simulink model "FMS"  (R2018b)
settings: configuration reference "fms_config" (kept outside this file)
values from neighbouring files (symbols this model uses):
  FMS_EXPORT = Simulink.Parameter(FMS_EXPORT_VALUE)    [fms_model_init.m]
  FMS_PARAM = Simulink.Parameter(FMS_PARAM_VALUE)    [fms_model_init.m]
undefined symbols (not defined in the file or in its folder): actuator_cmd, ax_cmd, ay_cmd, az_cmd, cmd_mask, ControlMode, ctrl_mode, DiscIntNeverNeededParam, ext_state, FMS_Cmd, FMS_CONST, home, mode, p_cmd, phi_cmd, PilotMode, psi_rate_cmd, q_cmd, r_cmd, reset, state, status, theta_cmd, throttle_cmd, timestamp, u_cmd, v_cmd, VehicleState, VehicleStatus, VTOLState, w_cmd, wp_consume, wp_current
libraries: simulink x141, FMT_Model_Lib x120, hdlsllib x13
(part 4 of 12)

== system FMS/FMS Commander/Commander/Arm/MC_Mode/SubMode/Takeoff/Climb Speed ==
  FMS_In : Inport
  Abs : Abs
  Abs1 : Abs
  Bus Selector : BusSelector  OutputSignals=INS_Out.h_R
  Bus Selector1 : BusSelector  OutputSignals=Cmd_In.cur_waypoint
  Bus Selector2 : BusSelector  OutputSignals=Cmd_In.sp_waypoint
  Compare To Constant : simulink/Logic and Bit Operations/Compare To Constant  relop=>  const=2.0  OutDataTypeStr=boolean
  Compare To Constant1 : simulink/Logic and Bit Operations/Compare To Constant  relop=>  const=2.0  OutDataTypeStr=boolean
  Gain : Gain  Gain=0.5
  Logical Operator : Logic  AllPortsSameDT=off  OutDataTypeStr=boolean
  Selector : Selector  InputPortWidth=3  IndexOptions=Index vector (dialog)  Indices=3  OutputSizes=1
  Selector1 : Selector  InputPortWidth=3  IndexOptions=Index vector (dialog)  Indices=3  OutputSizes=1
  Sum : Sum  Inputs=|+-
  Sum1 : Sum  Inputs=|+-
  Switch : Switch  Criteria=u2 ~= 0  Threshold=2
  TD : Subsystem
  Takeoff_Speed : Constant  Value=-FMS_PARAM.TAKEOFF_SPEED  OutDataTypeStr=Inherit: Inherit via back propagation
  w_cmd_mPs : Outport
  wires:
  Takeoff_Speed/1 -> Gain/1, Switch/1
  Sum/1 -> Abs/1
  Bus Selector/1 -> Sum1/2, Sum/1  "<h_R>"
  Switch/1 -> TD/1(v)
  FMS_In/1 -> Bus Selector2/1, Bus Selector/1, Bus Selector1/1
  Selector/1 -> Sum/2
  Bus Selector1/1 -> Selector/1  "<cur_waypoint>"
  Abs/1 -> Compare To Constant1/1
  Bus Selector2/1 -> Selector1/1  "<sp_waypoint>"
  Selector1/1 -> Sum1/1
  Sum1/1 -> Abs1/1
  Abs1/1 -> Compare To Constant/1
  Compare To Constant/1 -> Logical Operator/1
  Compare To Constant1/1 -> Logical Operator/2
  Logical Operator/1 -> Switch/2
  TD/1(v1) -> w_cmd_mPs/1
  Gain/1 -> Switch/3

== system FMS/FMS Commander/Commander/Arm/MC_Mode/SubMode/Takeoff/Track Position ==
  FMS_In : Inport
  Bus Selector : BusSelector  OutputSignals=INS_Out.psi
  Bus_Selection : Subsystem
  Constant : Constant  Value=0  OutDataTypeStr=Inherit: Inherit via back propagation
  Gain2 : Gain  Gain=FMS_PARAM.XY_P  OutDataTypeStr=single
  Multiply : Product  Multiplication=Matrix(*)
  Mux : Mux  Inputs=2
  Psi To DCM : FMT_Model_Lib/Transformation/Psi To DCM
      settings: SourceProductName=FMT Toolbox
  Saturation1 : Saturate  UpperLimit=FMS_PARAM.VEL_XY_LIM/5  LowerLimit=-FMS_PARAM.VEL_XY_LIM/5
  Selector : Selector  InputPortWidth=3  IndexOptions=Index vector (dialog)  Indices=[1 2]  OutputSizes=1
  Sum : Sum  Inputs=-+|
  Target Position : Subsystem
  uv_cmd_mPs : Outport
  wires:
  Saturation1/1 -> uv_cmd_mPs/1
  Bus Selector/1 -> Psi To DCM/1  "<psi>"
  Selector/1 -> Gain2/1
  Mux/1 -> Multiply/2
  Multiply/1 -> Selector/1
  Psi To DCM/1 -> Multiply/1  "M_CO"
  Constant/1 -> Mux/2
  FMS_In/1 -> Bus Selector/1, Target Position/1(FMS_In), Bus_Selection/1(FMS_In)
  Sum/1 -> Mux/1  "xy_err_R"
  Bus_Selection/1(xy_est_R) -> Sum/1  "xy_est_R"
  Gain2/1 -> Saturation1/1
  Target Position/1(xy_cmd_R) -> Sum/2

== system FMS/FMS Commander/Commander/Arm/BackwardTrans_Mode/Position Command/Controller/Hold Control/Fly_Direction ==
  FMS_In : Inport
  Bus Selector2 : BusSelector  OutputSignals=INS_Out.vn,INS_Out.ve,INS_Out.vd
  Bus Selector3 : BusSelector  OutputSignals=INS_Out.quat
  Multiply : Product  Multiplication=Matrix(*)
  Mux : Mux  Inputs=3
  Quaternion To DCM : FMT_Model_Lib/Quaternion/Quaternion To DCM
      settings: SourceProductName=FMT Toolbox
  Selector : Selector  InputPortWidth=3  IndexOptions=Index vector (dialog)  Indices=1  OutputSizes=1
  Sign : Signum
  sign : Outport
  wires:
  Bus Selector3/1 -> Quaternion To DCM/1  "<quat>"
  Multiply/1 -> Selector/1
  Bus Selector2/3 -> Mux/3  "<vd>"
  FMS_In/1 -> Bus Selector3/1, Bus Selector2/1
  Sign/1 -> sign/1
  Mux/1 -> Multiply/2
  Quaternion To DCM/1 -> Multiply/1
  Bus Selector2/2 -> Mux/2  "<ve>"
  Bus Selector2/1 -> Mux/1  "<vn>"
  Selector/1 -> Sign/1  "Vu"

== system FMS/FMS Commander/Commander/Arm/BackwardTrans_Mode/Position Command/Controller/Hold Control/L1_Reference_WP ==
  c : Inport
  p_0 : Inport  Port=2
  n : Inport  Port=3
  L1 : Inport  Port=4
  Compare To Zero : simulink/Logic and Bit Operations/Compare To Zero  relop=>  OutDataTypeStr=boolean
  OutRegionRefWP : MATLAB Function  TreatAsAtomicUnit=on
  SearchL1RefWP : MATLAB Function  TreatAsAtomicUnit=on
  Switch : Switch  Criteria=u2 > Threshold
  L1_WP : Outport
  wires:
  c/1 -> OutRegionRefWP/1(c), SearchL1RefWP/1(c)
  p_0/1 -> OutRegionRefWP/2(p0), SearchL1RefWP/2(p0)
  n/1 -> OutRegionRefWP/3(n), SearchL1RefWP/3(n)
  L1/1 -> SearchL1RefWP/4(L1)
  SearchL1RefWP/1(P) -> Switch/1
  SearchL1RefWP/2(t) -> Compare To Zero/1
  Compare To Zero/1 -> Switch/2
  OutRegionRefWP/1(P) -> Switch/3
  Switch/1 -> L1_WP/1

== system FMS/FMS Commander/Commander/Arm/BackwardTrans_Mode/Position Command/Controller/Hold Control/Lateral_Acceleration ==
  p_vehicle : Inport
  L1_WP : Inport  Port=2
  L1 : Inport  Port=3
  Vg : Inport  Port=4
  L1_Lateral_Acceleration : Subsystem
  Subtract : Sum  Inputs=+-
  ay_cmd_mPs2 : Outport
  wires:
  L1_WP/1 -> Subtract/1
  p_vehicle/1 -> Subtract/2
  L1/1 -> L1_Lateral_Acceleration/1(L1)
  Vg/1 -> L1_Lateral_Acceleration/2(Vg)
  Subtract/1 -> L1_Lateral_Acceleration/3(l1_path)
  L1_Lateral_Acceleration/1(l1_a_cmd) -> ay_cmd_mPs2/1

== system FMS/FMS Commander/Commander/Arm/BackwardTrans_Mode/Position Command/Controller/Hold Control/Path_Ray ==
  note: p(t) = p0 + t*n
  FMS_In : Inport
  Bus Selector1 : BusSelector  OutputSignals=INS_Out.x_R,INS_Out.y_R
  Bus Selector2 : BusSelector  OutputSignals=INS_Out.vn,INS_Out.ve
  Bus Selector3 : BusSelector  Commented=on  OutputSignals=INS_Out.psi
  Constant : Constant  Commented=on  Value=[1;0;0]  VectorParams1D=off  OutDataTypeStr=single
  Multiply : Product  Commented=on  Multiplication=Matrix(*)
  Mux : Mux  Inputs=2
  Mux1 : Mux  Inputs=2
  Psi To DCM : FMT_Model_Lib/Transformation/Psi To DCM  Commented=on
      settings: SourceProductName=FMT Toolbox
  Selector : Selector  Commented=on  InputPortWidth=3  IndexOptions=Index vector (dialog)  Indices=[1 2]  OutputSizes=1
  Terminator : Terminator  Commented=on
  Transpose : Math  Commented=on  Operator=transpose  SaturateOnIntegerOverflow=on
  Vector Normalize : FMT_Model_Lib/Math/Vector Normalize
      settings: SourceProductName=FMT Toolbox
  start_vel : Delay  DelayLength=1  InitialConditionSource=Input port
      settings: InputPortMap=u0,p4
  start_wp : Delay  DelayLength=1  InitialConditionSource=Input port
      settings: InputPortMap=u0,p4
  p_vehicle : Outport
  p_0 : Outport  Port=2
  n : Outport  Port=3
  wires:
  Bus Selector2/2 -> Mux1/2  "<ve>"
  Bus Selector1/2 -> Mux/2  "<y_R>"
  Mux/1 -> p_vehicle/1, start_wp/2
  start_wp/1 -> p_0/1, start_wp/1
  Bus Selector1/1 -> Mux/1  "<x_R>"
  start_vel/1 -> Vector Normalize/1, start_vel/1
  Bus Selector2/1 -> Mux1/1  "<vn>"
  Vector Normalize/1 -> n/1
  FMS_In/1 -> Bus Selector3/1, Bus Selector2/1, Bus Selector1/1
  Mux1/1 -> start_vel/2
  Bus Selector3/1 -> Psi To DCM/1  "<psi>"
  Psi To DCM/1 -> Transpose/1
  Transpose/1 -> Multiply/1
  Constant/1 -> Multiply/2
  Multiply/1 -> Selector/1
  Selector/1 -> Terminator/1

== system FMS/FMS Commander/Commander/Arm/BackwardTrans_Mode/Position Command/Controller/Hold Control/Velocity_Controller ==
  FMS_In : Inport
  Bus Selector : BusSelector  OutputSignals=INS_Out
  Constant : Constant  Value=0  OutDataTypeStr=Inherit: Inherit via back propagation
  Error : Subsystem
  PID_Controller : Subsystem
  ay_cmd_B_rad : Outport
  wires:
  FMS_In/1 -> Bus Selector/1
  Error/1(v_err_C_mPs) -> PID_Controller/1(uv_err_C_mPs)
  PID_Controller/1(accel_cmd_C) -> ay_cmd_B_rad/1
  Bus Selector/1 -> Error/1(INS_Out)  "<INS_Out>"
  Constant/1 -> PID_Controller/2(reset)

== system FMS/FMS Commander/Commander/Arm/BackwardTrans_Mode/Position Command/Controller/Move Control/DeadZone1 ==
  u : Inport
  Dead Zone : DeadZone  LowerValue=-th  UpperValue=th  SaturateOnIntegerOverflow=on
  Gain : Gain  Gain=1/(1-th)
  y : Outport
  wires:
  u/1 -> Dead Zone/1
  Dead Zone/1 -> Gain/1
  Gain/1 -> y/1

== system FMS/FMS Commander/Commander/Arm/BackwardTrans_Mode/Position Command/Controller/Move Control/TD ==
  v : Inport
  Integrator : DiscreteIntegrator  SampleTime=-1  ICPrevOutput=DiscIntNeverNeededParam  ICPrevScaledInput=DiscIntNeverNeededParam
  Integrator1 : DiscreteIntegrator  SampleTime=-1  ICPrevOutput=DiscIntNeverNeededParam  ICPrevScaledInput=DiscIntNeverNeededParam
  Subtract : Sum  Inputs=+-
  "fhan " : Subsystem  mask{r0=6*9.806, h0=0.05}
      mask DialogControl ParameterGroupVar Prompt: fhan(v1,v2,r0,h0)
  v1 : Outport
  wires:
  "fhan "/1(fhan) -> Integrator/1
  Subtract/1 -> "fhan "/1(v1)
  Integrator/1 -> Integrator1/1, "fhan "/2(v2)  "v2"
  v/1 -> Subtract/2
  Integrator1/1 -> Subtract/1, v1/1

== system FMS/FMS Commander/Commander/Arm/FW_Mode/Assist/Altitude/Altitude Command/Controller ==
  motion_state : Inport
  In Bus Element : Inport  Port=2  PortName=FMS_In
  In Bus Element1 : Inport  Port=2  PortName=FMS_In
  Hold Control : Subsystem  TreatAsAtomicUnit=on
  Merge : Merge
  Move Control : Subsystem  TreatAsAtomicUnit=on
  Saturation1 : Saturate  UpperLimit=FMS_PARAM.FW_VEL_Z_LIM  LowerLimit=-FMS_PARAM.FW_VEL_Z_LIM
  Switch Case : SwitchCase  CaseConditions={MotionState.Hold, [MotionState.Brake, MotionState.Move]}  ShowDefaultCase=off
  TD : Subsystem
  w_cmd_mPs : Outport
  wires:
  Move Control/1(w_cmd_mPs) -> Merge/2
  Hold Control/1(w_cmd_mPs) -> Merge/1
  In Bus Element/1 -> Hold Control/1(FMS_In)
  Switch Case/2 -> Move Control/Action
  Switch Case/1 -> Hold Control/Action
  motion_state/1 -> Switch Case/1
  Saturation1/1 -> TD/1(v)
  Merge/1 -> Saturation1/1
  In Bus Element1/1 -> Move Control/1(FMS_In)
  TD/1(v1) -> w_cmd_mPs/1

== system FMS/FMS Commander/Commander/Arm/FW_Mode/Assist/Altitude/Altitude Command/Detect Movement ==
  FMS_In : Inport
  Abs : Abs
  Abs1 : Abs
  Bus Selector : BusSelector  OutputSignals=Pilot_Cmd.stick_pitch,INS_Out.vd
  Compare To Constant : simulink/Logic and Bit Operations/Compare To Constant  relop=>  const=FMS_PARAM.PITCH_DZ  OutDataTypeStr=boolean
  Motion Status : Stateflow chart  TreatAsAtomicUnit=on
  motion_state : Outport
  wires:
  FMS_In/1 -> Bus Selector/1
  Abs1/1 -> Compare To Constant/1
  Motion Status/1(state) -> motion_state/1
  Compare To Constant/1 -> Motion Status/1(motion_req)
  Abs/1 -> Motion Status/2(speed)
  Bus Selector/1 -> Abs1/1  "<stick_pitch>"
  Bus Selector/2 -> Abs/1  "<vd>"

== system FMS/FMS Commander/Commander/Arm/FW_Mode/Assist/Altitude/Attitude Command/DeadZone ==
  u : Inport
  Dead Zone : DeadZone  LowerValue=-th  UpperValue=th  SaturateOnIntegerOverflow=on
  Gain : Gain  Gain=1/(1-th)
  y : Outport
  wires:
  Gain/1 -> y/1
  Dead Zone/1 -> Gain/1
  u/1 -> Dead Zone/1

== system FMS/FMS Commander/Commander/Arm/FW_Mode/Assist/Altitude/Attitude Command/TD ==
  v : Inport
  Integrator : DiscreteIntegrator  SampleTime=-1  ICPrevOutput=DiscIntNeverNeededParam  ICPrevScaledInput=DiscIntNeverNeededParam
  Integrator1 : DiscreteIntegrator  SampleTime=-1  ICPrevOutput=DiscIntNeverNeededParam  ICPrevScaledInput=DiscIntNeverNeededParam
  Subtract : Sum  Inputs=+-
  "fhan " : Subsystem  mask{r0=4*pi, h0=0.04}
      mask DialogControl ParameterGroupVar Prompt: fhan(v1,v2,r0,h0)
  v1 : Outport
  wires:
  "fhan "/1(fhan) -> Integrator/1
  Subtract/1 -> "fhan "/1(v1)
  Integrator/1 -> Integrator1/1, "fhan "/2(v2)  "v2"
  v/1 -> Subtract/2
  Integrator1/1 -> Subtract/1, v1/1

== system FMS/FMS Commander/Commander/Arm/FW_Mode/Assist/Altitude/Heading Command/DeadZone ==
  u : Inport
  Dead Zone : DeadZone  LowerValue=-th  UpperValue=th  SaturateOnIntegerOverflow=on
  Gain : Gain  Gain=1/(1-th)
  y : Outport
  wires:
  Gain/1 -> y/1
  Dead Zone/1 -> Gain/1
  u/1 -> Dead Zone/1

== system FMS/FMS Commander/Commander/Arm/FW_Mode/Assist/Altitude/Heading Command/TD ==
  v : Inport
  Integrator : DiscreteIntegrator  SampleTime=-1  ICPrevOutput=DiscIntNeverNeededParam  ICPrevScaledInput=DiscIntNeverNeededParam
  Integrator1 : DiscreteIntegrator  SampleTime=-1  ICPrevOutput=DiscIntNeverNeededParam  ICPrevScaledInput=DiscIntNeverNeededParam
  Subtract : Sum  Inputs=+-
  "fhan " : Subsystem  mask{r0=5*pi, h0=0.02}
      mask DialogControl ParameterGroupVar Prompt: fhan(v1,v2,r0,h0)
  v1 : Outport
  wires:
  "fhan "/1(fhan) -> Integrator/1
  Subtract/1 -> "fhan "/1(v1)
  Integrator/1 -> Integrator1/1, "fhan "/2(v2)  "v2"
  v/1 -> Subtract/2
  Integrator1/1 -> Subtract/1, v1/1

== system FMS/FMS Commander/Commander/Arm/FW_Mode/Assist/Altitude/Speed Command/StickToVelMapping ==
  In : Inport
  Constant : Constant  Value=max
  Constant1 : Constant  Value=mid
  Constant2 : Constant  Value=min
  Multiply : Product
  Multiply1 : Product
  Subtract : Sum  Inputs=+-
  Subtract1 : Sum  Inputs=+-
  Sum : Sum  Inputs=++|
  Sum1 : Sum  Inputs=++|
  Switch : Switch
  Out : Outport
  wires:
  In/1 -> Multiply1/1, Multiply/2, Switch/2
  Switch/1 -> Out/1
  Constant/1 -> Subtract/1
  Constant1/1 -> Sum1/1, Subtract1/1, Sum/1, Subtract/2
  Subtract/1 -> Multiply/1
  Multiply/1 -> Sum/2
  Sum/1 -> Switch/1
  Constant2/1 -> Subtract1/2
  Subtract1/1 -> Multiply1/2
  Multiply1/1 -> Sum1/2
  Sum1/1 -> Switch/3

== system FMS/FMS Commander/Commander/Arm/FW_Mode/Assist/Altitude/Speed Command/TD ==
  v : Inport
  Integrator : DiscreteIntegrator  SampleTime=-1  ICPrevOutput=DiscIntNeverNeededParam  ICPrevScaledInput=DiscIntNeverNeededParam
  Integrator1 : DiscreteIntegrator  SampleTime=-1  ICPrevOutput=DiscIntNeverNeededParam  ICPrevScaledInput=DiscIntNeverNeededParam
  Subtract : Sum  Inputs=+-
  "fhan " : Subsystem  mask{r0=8*9.806, h0=0.05}
      mask DialogControl ParameterGroupVar Prompt: fhan(v1,v2,r0,h0)
  v1 : Outport
  wires:
  Integrator1/1 -> v1/1, Subtract/1
  v/1 -> Subtract/2
  Integrator/1 -> "fhan "/2(v2), Integrator1/1  "v2"
  Subtract/1 -> "fhan "/1(v1)
  "fhan "/1(fhan) -> Integrator/1

== system FMS/FMS Commander/Commander/Arm/FW_Mode/Assist/Position/Altitude Command/Controller ==
  motion_state : Inport
  In Bus Element : Inport  Port=2  PortName=FMS_In
  In Bus Element1 : Inport  Port=2  PortName=FMS_In
  Hold Control : Subsystem  TreatAsAtomicUnit=on
  Merge : Merge
  Move Control : Subsystem  TreatAsAtomicUnit=on
  Saturation1 : Saturate  UpperLimit=FMS_PARAM.FW_VEL_Z_LIM  LowerLimit=-FMS_PARAM.FW_VEL_Z_LIM
  Switch Case : SwitchCase  CaseConditions={MotionState.Hold, [MotionState.Brake, MotionState.Move]}  ShowDefaultCase=off
  TD : Subsystem
  w_cmd_mPs : Outport
  wires:
  Move Control/1(w_cmd_mPs) -> Merge/2
  Hold Control/1(w_cmd_mPs) -> Merge/1
  In Bus Element/1 -> Hold Control/1(FMS_In)
  Switch Case/2 -> Move Control/Action
  Switch Case/1 -> Hold Control/Action
  motion_state/1 -> Switch Case/1
  Saturation1/1 -> TD/1(v)
  Merge/1 -> Saturation1/1
  In Bus Element1/1 -> Move Control/1(FMS_In)
  TD/1(v1) -> w_cmd_mPs/1

== system FMS/FMS Commander/Commander/Arm/FW_Mode/Assist/Position/Altitude Command/Detect Movement ==
  FMS_In : Inport
  Abs : Abs
  Abs1 : Abs
  Bus Selector : BusSelector  OutputSignals=Pilot_Cmd.stick_pitch,INS_Out.vd
  Compare To Constant : simulink/Logic and Bit Operations/Compare To Constant  relop=>  const=FMS_PARAM.PITCH_DZ  OutDataTypeStr=boolean
  Motion Status : Stateflow chart  TreatAsAtomicUnit=on
  motion_state : Outport
  wires:
  FMS_In/1 -> Bus Selector/1
  Abs1/1 -> Compare To Constant/1
  Motion Status/1(state) -> motion_state/1
  Compare To Constant/1 -> Motion Status/1(motion_req)
  Abs/1 -> Motion Status/2(speed)
  Bus Selector/1 -> Abs1/1  "<stick_pitch>"
  Bus Selector/2 -> Abs/1  "<vd>"

== system FMS/FMS Commander/Commander/Arm/FW_Mode/Assist/Position/Heading Command/DeadZone ==
  u : Inport
  Dead Zone : DeadZone  LowerValue=-th  UpperValue=th  SaturateOnIntegerOverflow=on
  Gain : Gain  Gain=1/(1-th)
  y : Outport
  wires:
  Gain/1 -> y/1
  Dead Zone/1 -> Gain/1
  u/1 -> Dead Zone/1

== system FMS/FMS Commander/Commander/Arm/FW_Mode/Assist/Position/Heading Command/TD ==
  v : Inport
  Integrator : DiscreteIntegrator  SampleTime=-1  ICPrevOutput=DiscIntNeverNeededParam  ICPrevScaledInput=DiscIntNeverNeededParam
  Integrator1 : DiscreteIntegrator  SampleTime=-1  ICPrevOutput=DiscIntNeverNeededParam  ICPrevScaledInput=DiscIntNeverNeededParam
  Subtract : Sum  Inputs=+-
  "fhan " : Subsystem  mask{r0=5*pi, h0=0.02}
      mask DialogControl ParameterGroupVar Prompt: fhan(v1,v2,r0,h0)
  v1 : Outport
  wires:
  "fhan "/1(fhan) -> Integrator/1
  Subtract/1 -> "fhan "/1(v1)
  Integrator/1 -> Integrator1/1, "fhan "/2(v2)  "v2"
  v/1 -> Subtract/2
  Integrator1/1 -> Subtract/1, v1/1

== system FMS/FMS Commander/Commander/Arm/FW_Mode/Assist/Position/Position Command/Controller ==
  motion_state : Inport
  In Bus Element : Inport  Port=2  PortName=FMS_In
  In Bus Element1 : Inport  Port=2  PortName=FMS_In
  Hold Control : Subsystem  TreatAsAtomicUnit=on
  Merge : Merge
  Move Control : Subsystem  TreatAsAtomicUnit=on
  Saturation1 : Saturate  UpperLimit=FMS_PARAM.FW_ACC_Y_LIM  LowerLimit=-FMS_PARAM.FW_ACC_Y_LIM
  Switch Case : SwitchCase  CaseConditions={MotionState.Hold, [MotionState.Brake, MotionState.Move]}  ShowDefaultCase=off
  ay_cmd_mPs2 : Outport
  wires:
  Move Control/1(ay_cmd_mPs2) -> Merge/2
  Hold Control/1(ay_cmd_mPs2) -> Merge/1
  In Bus Element/1 -> Hold Control/1(FMS_In)
  Switch Case/2 -> Move Control/Action
  Switch Case/1 -> Hold Control/Action
  motion_state/1 -> Switch Case/1
  Saturation1/1 -> ay_cmd_mPs2/1
  Merge/1 -> Saturation1/1
  In Bus Element1/1 -> Move Control/1(FMS_In)

== system FMS/FMS Commander/Commander/Arm/FW_Mode/Assist/Position/Position Command/Detect Movement ==
  FMS_In : Inport
  Abs : Abs
  Abs1 : Abs
  Abs2 : Abs
  Bus Selector1 : BusSelector  OutputSignals=Pilot_Cmd.stick_roll,Pilot_Cmd.stick_yaw
  Bus Selector2 : BusSelector  OutputSignals=INS_Out.psi,INS_Out.vn,INS_Out.ve,INS_Out.vd
  Compare To Constant : simulink/Logic and Bit Operations/Compare To Constant  relop=>  const=FMS_PARAM.ROLL_DZ  OutDataTypeStr=boolean
  Compare To Constant1 : simulink/Logic and Bit Operations/Compare To Constant  relop=>  const=FMS_PARAM.YAW_DZ  OutDataTypeStr=boolean
  Logical Operator : Logic  Operator=OR  AllPortsSameDT=off  OutDataTypeStr=boolean
  Motion State : Stateflow chart  TreatAsAtomicUnit=on
  Multiply : Product  Multiplication=Matrix(*)
  Mux : Mux  Inputs=3
  Psi To DCM : FMT_Model_Lib/Transformation/Psi To DCM
      settings: SourceProductName=FMT Toolbox
  Selector : Selector  InputPortWidth=3  IndexOptions=Index vector (dialog)  Indices=1  OutputSizes=1
  motion_state : Outport
  wires:
  FMS_In/1 -> Bus Selector2/1, Bus Selector1/1
  Abs1/1 -> Compare To Constant/1
  Motion State/1(state) -> motion_state/1  "pos_ms"
  Abs/1 -> Motion State/2(speed)
  Bus Selector1/1 -> Abs1/1  "<stick_roll>"
  Bus Selector2/1 -> Psi To DCM/1  "<psi>"
  Bus Selector2/2 -> Mux/1  "<vn>"
  Bus Selector2/3 -> Mux/2  "<ve>"
  Bus Selector2/4 -> Mux/3  "<vd>"
  Psi To DCM/1 -> Multiply/1
  Multiply/1 -> Selector/1
  Selector/1 -> Abs/1
  Mux/1 -> Multiply/2
  Bus Selector1/2 -> Abs2/1  "<stick_yaw>"
  Abs2/1 -> Compare To Constant1/1
  Compare To Constant/1 -> Logical Operator/1
  Compare To Constant1/1 -> Logical Operator/2
  Logical Operator/1 -> Motion State/1(motion_req)

== system FMS/FMS Commander/Commander/Arm/FW_Mode/Assist/Position/Speed Command/StickToVelMapping ==
  In : Inport
  Constant : Constant  Value=max
  Constant1 : Constant  Value=mid
  Constant2 : Constant  Value=min
  Multiply : Product
  Multiply1 : Product
  Subtract : Sum  Inputs=+-
  Subtract1 : Sum  Inputs=+-
  Sum : Sum  Inputs=++|
  Sum1 : Sum  Inputs=++|
  Switch : Switch
  Out : Outport
  wires:
  In/1 -> Multiply1/1, Multiply/2, Switch/2
  Switch/1 -> Out/1
  Constant/1 -> Subtract/1
  Constant1/1 -> Sum1/1, Subtract1/1, Sum/1, Subtract/2
  Subtract/1 -> Multiply/1
  Multiply/1 -> Sum/2
  Sum/1 -> Switch/1
  Constant2/1 -> Subtract1/2
  Subtract1/1 -> Multiply1/2
  Multiply1/1 -> Sum1/2
  Sum1/1 -> Switch/3

== system FMS/FMS Commander/Commander/Arm/FW_Mode/Assist/Position/Speed Command/TD ==
  v : Inport
  Integrator : DiscreteIntegrator  SampleTime=-1  ICPrevOutput=DiscIntNeverNeededParam  ICPrevScaledInput=DiscIntNeverNeededParam
  Integrator1 : DiscreteIntegrator  SampleTime=-1  ICPrevOutput=DiscIntNeverNeededParam  ICPrevScaledInput=DiscIntNeverNeededParam
  Subtract : Sum  Inputs=+-
  "fhan " : Subsystem  mask{r0=8*9.806, h0=0.05}
      mask DialogControl ParameterGroupVar Prompt: fhan(v1,v2,r0,h0)
  v1 : Outport
  wires:
  Integrator1/1 -> v1/1, Subtract/1
  v/1 -> Subtract/2
  Integrator/1 -> "fhan "/2(v2), Integrator1/1  "v2"
  Subtract/1 -> "fhan "/1(v1)
  "fhan "/1(fhan) -> Integrator/1

== system FMS/FMS Commander/Commander/Arm/FW_Mode/Assist/Stabilize/Attitude Command/DeadZone ==
  u : Inport
  Dead Zone : DeadZone  LowerValue=-th  UpperValue=th  SaturateOnIntegerOverflow=on
  Gain : Gain  Gain=1/(1-th)
  y : Outport
  wires:
  Gain/1 -> y/1
  Dead Zone/1 -> Gain/1
  u/1 -> Dead Zone/1

== system FMS/FMS Commander/Commander/Arm/FW_Mode/Assist/Stabilize/Attitude Command/DeadZone2 ==
  u : Inport
  Dead Zone : DeadZone  LowerValue=-th  UpperValue=th  SaturateOnIntegerOverflow=on
  Gain : Gain  Gain=1/(1-th)
  y : Outport
  wires:
  u/1 -> Dead Zone/1
  Dead Zone/1 -> Gain/1
  Gain/1 -> y/1

== system FMS/FMS Commander/Commander/Arm/FW_Mode/Assist/Stabilize/Attitude Command/Phi_CMD_TD ==
  v : Inport
  Integrator : DiscreteIntegrator  SampleTime=-1  ICPrevOutput=DiscIntNeverNeededParam  ICPrevScaledInput=DiscIntNeverNeededParam
  Integrator1 : DiscreteIntegrator  SampleTime=-1  ICPrevOutput=DiscIntNeverNeededParam  ICPrevScaledInput=DiscIntNeverNeededParam
  Subtract : Sum  Inputs=+-
  "fhan " : Subsystem  mask{r0=4*pi, h0=0.04}
      mask DialogControl ParameterGroupVar Prompt: fhan(v1,v2,r0,h0)
  v1 : Outport
  wires:
  "fhan "/1(fhan) -> Integrator/1
  Subtract/1 -> "fhan "/1(v1)
  Integrator/1 -> Integrator1/1, "fhan "/2(v2)  "v2"
  v/1 -> Subtract/2
  Integrator1/1 -> Subtract/1, v1/1

== system FMS/FMS Commander/Commander/Arm/FW_Mode/Assist/Stabilize/Attitude Command/Theta_CMD_TD ==
  v : Inport
  Integrator : DiscreteIntegrator  SampleTime=-1  ICPrevOutput=DiscIntNeverNeededParam  ICPrevScaledInput=DiscIntNeverNeededParam
  Integrator1 : DiscreteIntegrator  SampleTime=-1  ICPrevOutput=DiscIntNeverNeededParam  ICPrevScaledInput=DiscIntNeverNeededParam
  Subtract : Sum  Inputs=+-
  "fhan " : Subsystem  mask{r0=4*pi, h0=0.04}
      mask DialogControl ParameterGroupVar Prompt: fhan(v1,v2,r0,h0)
  v1 : Outport
  wires:
  Integrator1/1 -> v1/1, Subtract/1
  v/1 -> Subtract/2
  Integrator/1 -> Integrator1/1, "fhan "/2(v2)  "v2"
  Subtract/1 -> "fhan "/1(v1)
  "fhan "/1(fhan) -> Integrator/1

== system FMS/FMS Commander/Commander/Arm/FW_Mode/Assist/Stabilize/Heading Command/DeadZone ==
  u : Inport
  Dead Zone : DeadZone  LowerValue=-th  UpperValue=th  SaturateOnIntegerOverflow=on
  Gain : Gain  Gain=1/(1-th)
  y : Outport
  wires:
  Gain/1 -> y/1
  Dead Zone/1 -> Gain/1
  u/1 -> Dead Zone/1

== system FMS/FMS Commander/Commander/Arm/FW_Mode/Assist/Stabilize/Heading Command/TD ==
  v : Inport
  Integrator : DiscreteIntegrator  SampleTime=-1  ICPrevOutput=DiscIntNeverNeededParam  ICPrevScaledInput=DiscIntNeverNeededParam
  Integrator1 : DiscreteIntegrator  SampleTime=-1  ICPrevOutput=DiscIntNeverNeededParam  ICPrevScaledInput=DiscIntNeverNeededParam
  Subtract : Sum  Inputs=+-
  "fhan " : Subsystem  mask{r0=5*pi, h0=0.02}
      mask DialogControl ParameterGroupVar Prompt: fhan(v1,v2,r0,h0)
  v1 : Outport
  wires:
  "fhan "/1(fhan) -> Integrator/1
  Subtract/1 -> "fhan "/1(v1)
  Integrator/1 -> Integrator1/1, "fhan "/2(v2)  "v2"
  v/1 -> Subtract/2
  Integrator1/1 -> Subtract/1, v1/1

== system FMS/FMS Commander/Commander/Arm/FW_Mode/Auto/Mission/Mission_SubSystem/Altitude Control ==
  FMS_In : Inport
  Bus Selector3 : BusSelector  OutputSignals=INS_Out.h_R
  Gain : Gain  Gain=FMS_PARAM.FW_Z_P
  Saturation1 : Saturate  UpperLimit=FMS_PARAM.FW_VEL_Z_LIM  LowerLimit=-FMS_PARAM.FW_VEL_Z_LIM
  Sum2 : Sum  Inputs=|+-
  Target Height : Subsystem
  w_cmd_mPs : Outport
  wires:
  FMS_In/1 -> Bus Selector3/1, Target Height/1(FMS_In)
  Bus Selector3/1 -> Sum2/1  "<h_R>"
  Sum2/1 -> Gain/1
  Gain/1 -> Saturation1/1
  Target Height/1(h_R_sp) -> Sum2/2  "h_R_sp"
  Saturation1/1 -> w_cmd_mPs/1

== system FMS/FMS Commander/Commander/Arm/FW_Mode/Auto/Mission/Mission_SubSystem/Cruise_Speed ==
  FMS_In : Inport
  Bus Selector : BusSelector  OutputSignals=Cmd_In.set_speed
  Constant4 : Constant  Value=FMS_PARAM.FW_CRUISE_SPEED
  Saturation : Saturate  UpperLimit=FMS_PARAM.FW_SPEED_MAX  LowerLimit=FMS_PARAM.FW_SPEED_MIN
  Switch : Switch  Criteria=u2 > Threshold
  TD : Subsystem
  u_cmd : Outport
  wires:
  FMS_In/1 -> Bus Selector/1
  Bus Selector/1 -> Switch/1, Switch/2  "<set_speed>"
  Constant4/1 -> Switch/3
  TD/1(v1) -> Saturation/1
  Switch/1 -> TD/1(v)
  Saturation/1 -> u_cmd/1

== system FMS/FMS Commander/Commander/Arm/FW_Mode/Auto/Mission/Mission_SubSystem/Position Command ==
  FMS_In : Inport
  L1 Control : Subsystem
  WayPoints : Subsystem
  ay_cmd_mPs2 : Outport
  wires:
  FMS_In/1 -> L1 Control/4(FMS_In), WayPoints/1(FMS_In)
  L1 Control/1(ay_cmd_mPs2) -> ay_cmd_mPs2/1
  WayPoints/2(p2) -> L1 Control/2(p2)
  WayPoints/3(p3) -> L1 Control/3(p3)
  WayPoints/1(p1) -> L1 Control/1(p1)

== system FMS/FMS Commander/Commander/Arm/FW_Mode/SubMode/Hold/Altitude_Hold/Bus_Selection ==
  FMS_In : Inport
  Bus Selector2 : BusSelector  OutputSignals=INS_Out.h_R
  Gain : Gain  Gain=-1
  z_R_m : Outport
  wires:
  Gain/1 -> z_R_m/1
  Bus Selector2/1 -> Gain/1  "<h_R>"
  FMS_In/1 -> Bus Selector2/1

== system FMS/FMS Commander/Commander/Arm/FW_Mode/SubMode/Hold/Loiter_Control/L1 Reference WP ==
  P_Vehicle : Inport
  P_0 : Inport  Port=2
  n : Inport  Port=3
  R : Inport  Port=4
  L1 : Inport  Port=5
  Compare To Constant : simulink/Logic and Bit Operations/Compare To Constant  relop=>  const=0  OutDataTypeStr=boolean
  Gain : Gain  Gain=0.5
  Max : MinMax  Function=max  Inputs=2
  OutRegionRegWP : MATLAB Function  TreatAsAtomicUnit=on
  Reshape : Reshape  OutputDimensionality=Customize  OutputDimensions=[2,1]
  Reshape1 : Reshape  OutputDimensionality=Column vector (2-D)
  Reshape2 : Reshape  OutputDimensionality=Column vector (2-D)
  Reshape3 : Reshape  OutputDimensionality=Column vector (2-D)
  SearchL1RefWP : MATLAB Function  TreatAsAtomicUnit=on
  Switch : Switch  Criteria=u2 > Threshold
  L1_WP : Outport
  wires:
  Reshape/1 -> L1_WP/1
  Compare To Constant/1 -> Switch/2
  SearchL1RefWP/2(n) -> Compare To Constant/1
  OutRegionRegWP/1(P) -> Switch/3
  Switch/1 -> Reshape/1
  SearchL1RefWP/1(P) -> Switch/1
  P_0/1 -> Reshape1/1
  P_Vehicle/1 -> Reshape2/1
  Max/1 -> OutRegionRegWP/3(R), SearchL1RefWP/3(R)
  L1/1 -> Gain/1, OutRegionRegWP/4(L1), SearchL1RefWP/4(L1)
  Reshape1/1 -> OutRegionRegWP/1(P0), SearchL1RefWP/1(P_0)
  Reshape2/1 -> OutRegionRegWP/2(P_Vehicle), SearchL1RefWP/2(P_Vehicle)
  n/1 -> Reshape3/1
  Reshape3/1 -> OutRegionRegWP/5(n)
  R/1 -> Max/1
  Gain/1 -> Max/2

== system FMS/FMS Commander/Commander/Arm/FW_Mode/SubMode/Hold/Loiter_Control/L1_Core ==
  p_vehicle : Inport
  L1_WP : Inport  Port=2
  L1 : Inport  Port=3
  Vg : Inport  Port=4
  L1_Lateral_Acceleration : Subsystem
  Subtract : Sum  Inputs=+-
  ay_cmd_mPs2 : Outport
  wires:
  L1_WP/1 -> Subtract/1
  p_vehicle/1 -> Subtract/2
  L1/1 -> L1_Lateral_Acceleration/1(L1)
  Vg/1 -> L1_Lateral_Acceleration/2(Vg)
  Subtract/1 -> L1_Lateral_Acceleration/3(l1_path)
  L1_Lateral_Acceleration/1(l1_a_cmd) -> ay_cmd_mPs2/1

== system FMS/FMS Commander/Commander/Arm/FW_Mode/SubMode/Hold/Loiter_Control/Reference_Point ==
  FMS_In : Inport
  Bus Selector1 : BusSelector  OutputSignals=Cmd_In.sp_waypoint
  Bus Selector2 : BusSelector  OutputSignals=INS_Out.vn,INS_Out.ve
  Bus Selector3 : BusSelector  OutputSignals=INS_Out.x_R,INS_Out.y_R
  Mux1 : Mux  Inputs=2
  Mux2 : Mux  Inputs=2
  Selector : Selector  InputPortWidth=3  IndexOptions=Index vector (dialog)  Indices=[1 2]  OutputSizes=1
  Vector Normalize : FMT_Model_Lib/Math/Vector Normalize
      settings: SourceProductName=FMT Toolbox
  start_vel : Delay  DelayLength=1  InitialConditionSource=Input port
      settings: InputPortMap=u0,p4
  p_vehicle : Outport
  p_0 : Outport  Port=2
  n : Outport  Port=3
  wires:
  Bus Selector2/2 -> Mux1/2  "<ve>"
  start_vel/1 -> Vector Normalize/1, start_vel/1
  Bus Selector2/1 -> Mux1/1  "<vn>"
  Vector Normalize/1 -> n/1
  FMS_In/1 -> Bus Selector3/1, Bus Selector2/1, Bus Selector1/1
  Mux1/1 -> start_vel/2
  Bus Selector3/1 -> Mux2/1  "<x_R>"
  Bus Selector3/2 -> Mux2/2  "<y_R>"
  Mux2/1 -> p_vehicle/1
  Bus Selector1/1 -> Selector/1  "<sp_waypoint>"
  Selector/1 -> p_0/1

== system FMS/FMS Commander/Commander/Arm/FW_Mode/SubMode/Return/Altitude Control/Target Height ==
  FMS_In : Inport
  Add : Sum
  Bus Selector : BusSelector  OutputSignals=Cmd_In.sp_waypoint,Cmd_In.cur_waypoint
  Bus Selector1 : BusSelector  OutputSignals=INS_Out.x_R,INS_Out.y_R
  Bus Selector2 : BusSelector  OutputSignals=Cmd_In.cur_waypoint,Cmd_In.sp_waypoint
  Divide : Product  Inputs=*/
  Multiply : Product
  Mux : Mux  Inputs=2
  Saturation : Saturate  UpperLimit=1  LowerLimit=0
  Selector : Selector  InputPortWidth=3  IndexOptions=Index vector (dialog)  Indices=3  OutputSizes=1
  Selector1 : Selector  InputPortWidth=3  IndexOptions=Index vector (dialog)  Indices=3  OutputSizes=1
  Selector2 : Selector  InputPortWidth=3  IndexOptions=Index vector (dialog)  Indices=[1 2]  OutputSizes=1
  Selector3 : Selector  InputPortWidth=3  IndexOptions=Index vector (dialog)  Indices=[1 2]  OutputSizes=1
  Subtract : Sum  Inputs=+-
  Sum : Sum  Inputs=|+-
  Sum1 : Sum  Inputs=-+|
  Vector Modulus : FMT_Model_Lib/Math/Vector Modulus
      settings: SourceProductName=FMT Toolbox
  Vector Modulus1 : FMT_Model_Lib/Math/Vector Modulus
      settings: SourceProductName=FMT Toolbox
  h_R_sp : Outport
  wires:
  Multiply/1 -> Add/2
  Bus Selector1/1 -> Mux/1  "<x_R>"
  Bus Selector/1 -> Selector1/1  "<sp_waypoint>"
  Vector Modulus1/1 -> Divide/2
  Sum1/1 -> Vector Modulus1/1
  Sum/1 -> Vector Modulus/1
  Selector2/1 -> Sum1/1, Sum/2
  FMS_In/1 -> Bus Selector2/1, Bus Selector1/1, Bus Selector/1
  Bus Selector2/2 -> Selector3/1  "<sp_waypoint>"
  Vector Modulus/1 -> Divide/1
  Bus Selector1/2 -> Mux/2  "<y_R>"
  Bus Selector2/1 -> Selector2/1  "<cur_waypoint>"
  Selector1/1 -> Subtract/1
  Mux/1 -> Sum/1
  Subtract/1 -> Multiply/1
  Divide/1 -> Saturation/1
  Selector3/1 -> Sum1/2
  Bus Selector/2 -> Selector/1  "<cur_waypoint>"
  Selector/1 -> Add/1, Subtract/2
  Saturation/1 -> Multiply/2
  Add/1 -> h_R_sp/1

== system FMS/FMS Commander/Commander/Arm/FW_Mode/SubMode/Return/Position Command/L1 Control ==
  p1 : Inport
  p2 : Inport  Port=2
  p3 : Inport  Port=3
  FMS_In : Inport  Port=4
  Bus Selector1 : BusSelector  OutputSignals=INS_Out.vn,INS_Out.ve
  L1 : Constant  Value=FMS_PARAM.FW_L1  OutDataTypeStr=single
  L1 Reference WP : Subsystem
  L1_Core : Subsystem
  Mux : Mux  Inputs=2
  Saturation1 : Saturate  UpperLimit=FMS_PARAM.FW_ACC_Y_LIM  LowerLimit=-FMS_PARAM.FW_ACC_Y_LIM
  ay_cmd_mPs2 : Outport
  wires:
  p3/1 -> L1_Core/1(p_vehicle), L1 Reference WP/3(P3)
  p2/1 -> L1 Reference WP/2(P2)
  p1/1 -> L1 Reference WP/1(P1)
  L1/1 -> L1_Core/3(L1), L1 Reference WP/4(L1)
  L1 Reference WP/1(L1_WP) -> L1_Core/2(L1_WP)  "L1_WP"
  Mux/1 -> L1_Core/4(Vg)
  Bus Selector1/1 -> Mux/1  "<vn>"
  Bus Selector1/2 -> Mux/2  "<ve>"
  FMS_In/1 -> Bus Selector1/1
  L1_Core/1(ay_cmd_mPs2) -> Saturation1/1
  Saturation1/1 -> ay_cmd_mPs2/1

== system FMS/FMS Commander/Commander/Arm/FW_Mode/SubMode/Return/Position Command/WayPoints ==
  note: P1: path start point
      | P2: path end point
      | P3: vehicle point
  FMS_In : Inport
  Bus Selector : BusSelector  OutputSignals=INS_Out.x_R,INS_Out.y_R
  Bus Selector1 : BusSelector  OutputSignals=Cmd_In.sp_waypoint
  Bus Selector2 : BusSelector  OutputSignals=Cmd_In.cur_waypoint
  Mux : Mux  Inputs=2
  Reshape : Reshape  OutputDimensionality=Customize  OutputDimensions=[2,1]
  Reshape1 : Reshape  OutputDimensionality=Customize  OutputDimensions=[2,1]
  Reshape2 : Reshape  OutputDimensionality=Customize  OutputDimensions=[2,1]
  Selector : Selector  InputPortWidth=3  IndexOptions=Index vector (dialog)  Indices=[1 2]  OutputSizes=1
  Selector1 : Selector  InputPortWidth=3  IndexOptions=Index vector (dialog)  Indices=[1 2]  OutputSizes=1
  p1 : Outport
  p2 : Outport  Port=2
  p3 : Outport  Port=3
  wires:
  Reshape2/1 -> p3/1
  Reshape1/1 -> p1/1
  Reshape/1 -> p2/1
  Bus Selector/2 -> Mux/2  "<y_R>"
  Bus Selector/1 -> Mux/1  "<x_R>"
  Mux/1 -> Reshape2/1
  Bus Selector1/1 -> Selector/1  "<sp_waypoint>"
  Selector/1 -> Reshape/1
  Selector1/1 -> Reshape1/1
  Bus Selector2/1 -> Selector1/1  "<cur_waypoint>"
  FMS_In/1 -> Bus Selector2/1, Bus Selector1/1, Bus Selector/1

== system FMS/FMS Commander/Commander/Arm/FW_Mode/SubMode/Takeoff/Altitude Control/Target Height ==
  FMS_In : Inport
  Add : Sum
  Bus Selector : BusSelector  OutputSignals=Cmd_In.sp_waypoint,Cmd_In.cur_waypoint
  Bus Selector1 : BusSelector  OutputSignals=INS_Out.x_R,INS_Out.y_R
  Bus Selector2 : BusSelector  OutputSignals=Cmd_In.cur_waypoint,Cmd_In.sp_waypoint
  Divide : Product  Inputs=*/
  Multiply : Product
  Mux : Mux  Inputs=2
  Saturation : Saturate  UpperLimit=1  LowerLimit=0
  Selector : Selector  InputPortWidth=3  IndexOptions=Index vector (dialog)  Indices=3  OutputSizes=1
  Selector1 : Selector  InputPortWidth=3  IndexOptions=Index vector (dialog)  Indices=3  OutputSizes=1
  Selector2 : Selector  InputPortWidth=3  IndexOptions=Index vector (dialog)  Indices=[1 2]  OutputSizes=1
  Selector3 : Selector  InputPortWidth=3  IndexOptions=Index vector (dialog)  Indices=[1 2]  OutputSizes=1
  Subtract : Sum  Inputs=+-
  Sum : Sum  Inputs=|+-
  Sum1 : Sum  Inputs=-+|
  Vector Modulus : FMT_Model_Lib/Math/Vector Modulus
      settings: SourceProductName=FMT Toolbox
  Vector Modulus1 : FMT_Model_Lib/Math/Vector Modulus
      settings: SourceProductName=FMT Toolbox
  h_R_sp : Outport
  wires:
  Multiply/1 -> Add/2
  Bus Selector1/1 -> Mux/1  "<x_R>"
  Bus Selector/1 -> Selector1/1  "<sp_waypoint>"
  Vector Modulus1/1 -> Divide/2
  Sum1/1 -> Vector Modulus1/1
  Sum/1 -> Vector Modulus/1
  Selector2/1 -> Sum1/1, Sum/2
  FMS_In/1 -> Bus Selector2/1, Bus Selector1/1, Bus Selector/1
  Bus Selector2/2 -> Selector3/1  "<sp_waypoint>"
  Vector Modulus/1 -> Divide/1
  Bus Selector1/2 -> Mux/2  "<y_R>"
  Bus Selector2/1 -> Selector2/1  "<cur_waypoint>"
  Selector1/1 -> Subtract/1
  Mux/1 -> Sum/1
  Subtract/1 -> Multiply/1
  Divide/1 -> Saturation/1
  Selector3/1 -> Sum1/2
  Bus Selector/2 -> Selector/1  "<cur_waypoint>"
  Selector/1 -> Add/1, Subtract/2
  Saturation/1 -> Multiply/2
  Add/1 -> h_R_sp/1

== system FMS/FMS Commander/Commander/Arm/FW_Mode/SubMode/Takeoff/Position Command/L1 Control ==
  p1 : Inport
  p2 : Inport  Port=2
  p3 : Inport  Port=3
  FMS_In : Inport  Port=4
  Bus Selector1 : BusSelector  OutputSignals=INS_Out.vn,INS_Out.ve
  L1 : Constant  Value=FMS_PARAM.FW_L1  OutDataTypeStr=single
  L1 Reference WP : Subsystem
  L1_Core : Subsystem
  Mux : Mux  Inputs=2
  Saturation1 : Saturate  UpperLimit=FMS_PARAM.FW_ACC_Y_LIM  LowerLimit=-FMS_PARAM.FW_ACC_Y_LIM
  ay_cmd_mPs2 : Outport
  wires:
  p3/1 -> L1_Core/1(p_vehicle), L1 Reference WP/3(P3)
  p2/1 -> L1 Reference WP/2(P2)
  p1/1 -> L1 Reference WP/1(P1)
  L1/1 -> L1_Core/3(L1), L1 Reference WP/4(L1)
  L1 Reference WP/1(L1_WP) -> L1_Core/2(L1_WP)  "L1_WP"
  Mux/1 -> L1_Core/4(Vg)
  Bus Selector1/1 -> Mux/1  "<vn>"
  Bus Selector1/2 -> Mux/2  "<ve>"
  FMS_In/1 -> Bus Selector1/1
  L1_Core/1(ay_cmd_mPs2) -> Saturation1/1
  Saturation1/1 -> ay_cmd_mPs2/1

== system FMS/FMS Commander/Commander/Arm/FW_Mode/SubMode/Takeoff/Position Command/WayPoints ==
  note: P1: path start point
      | P2: path end point
      | P3: vehicle point
  FMS_In : Inport
  Bus Selector : BusSelector  OutputSignals=INS_Out.x_R,INS_Out.y_R
  Bus Selector1 : BusSelector  OutputSignals=Cmd_In.sp_waypoint
  Bus Selector2 : BusSelector  OutputSignals=Cmd_In.cur_waypoint
  Mux : Mux  Inputs=2
  Reshape : Reshape  OutputDimensionality=Customize  OutputDimensions=[2,1]
  Reshape1 : Reshape  OutputDimensionality=Customize  OutputDimensions=[2,1]
  Reshape2 : Reshape  OutputDimensionality=Customize  OutputDimensions=[2,1]
  Selector : Selector  InputPortWidth=3  IndexOptions=Index vector (dialog)  Indices=[1 2]  OutputSizes=1
  Selector1 : Selector  InputPortWidth=3  IndexOptions=Index vector (dialog)  Indices=[1 2]  OutputSizes=1
  p1 : Outport
  p2 : Outport  Port=2
  p3 : Outport  Port=3
  wires:
  Reshape2/1 -> p3/1
  Reshape1/1 -> p1/1
  Reshape/1 -> p2/1
  Bus Selector/2 -> Mux/2  "<y_R>"
  Bus Selector/1 -> Mux/1  "<x_R>"
  Mux/1 -> Reshape2/1
  FMS_In/1 -> Bus Selector2/1, Bus Selector1/1, Bus Selector/1
  Bus Selector1/1 -> Selector/1  "<sp_waypoint>"
  Selector/1 -> Reshape/1
  Bus Selector2/1 -> Selector1/1  "<cur_waypoint>"
  Selector1/1 -> Reshape1/1

== system FMS/FMS Commander/Commander/Arm/MC_Mode/Assist/Altitude/Altitude Command/Controller ==
  motion_state : Inport
  In Bus Element : Inport  Port=2  PortName=FMS_In
  In Bus Element1 : Inport  Port=2  PortName=FMS_In
  Brake Control : Subsystem  TreatAsAtomicUnit=on
  Hold Control : Subsystem  TreatAsAtomicUnit=on
  Merge : Merge  Inputs=3
  Move Control : Subsystem  TreatAsAtomicUnit=on
  Saturation1 : Saturate  UpperLimit=FMS_PARAM.VEL_Z_LIM  LowerLimit=-FMS_PARAM.VEL_Z_LIM
  Switch Case : SwitchCase  CaseConditions={MotionState.Hold, MotionState.Brake, MotionState.Move}  ShowDefaultCase=off
  w_cmd_mPs : Outport
  wires:
  Move Control/1(w_cmd_mPs) -> Merge/3
  Brake Control/1(psi_rate_cmd_radPs) -> Merge/2
  Hold Control/1(w_cmd_mPs) -> Merge/1
  In Bus Element/1 -> Hold Control/1(FMS_In)
  Switch Case/2 -> Brake Control/Action
  Switch Case/1 -> Hold Control/Action
  motion_state/1 -> Switch Case/1
  Saturation1/1 -> w_cmd_mPs/1
  Merge/1 -> Saturation1/1
  Switch Case/3 -> Move Control/Action
  In Bus Element1/1 -> Move Control/1(FMS_In)

== system FMS/FMS Commander/Commander/Arm/MC_Mode/Assist/Altitude/Altitude Command/Detect Movement ==
  FMS_In : Inport
  Abs : Abs
  Abs1 : Abs
  Bus Selector : BusSelector  OutputSignals=Pilot_Cmd.stick_throttle,INS_Out.vd
  Compare To Constant : simulink/Logic and Bit Operations/Compare To Constant  relop=>  const=FMS_PARAM.THROTTLE_DZ  OutDataTypeStr=boolean
  Motion Status : Stateflow chart  TreatAsAtomicUnit=on
  motion_state : Outport
  wires:
  FMS_In/1 -> Bus Selector/1
  Abs1/1 -> Compare To Constant/1
  Motion Status/1(state) -> motion_state/1
  Compare To Constant/1 -> Motion Status/1(motion_req)
  Abs/1 -> Motion Status/2(speed)
  Bus Selector/1 -> Abs1/1  "<stick_throttle>"
  Bus Selector/2 -> Abs/1  "<vd>"

== system FMS/FMS Commander/Commander/Arm/MC_Mode/Assist/Altitude/Attitude Command/DeadZone ==
  u : Inport
  Dead Zone : DeadZone  LowerValue=-th  UpperValue=th  SaturateOnIntegerOverflow=on
  Gain : Gain  Gain=1/(1-th)
  y : Outport
  wires:
  Gain/1 -> y/1
  Dead Zone/1 -> Gain/1
  u/1 -> Dead Zone/1

== system FMS/FMS Commander/Commander/Arm/MC_Mode/Assist/Altitude/Attitude Command/DeadZone2 ==
  u : Inport
  Dead Zone : DeadZone  LowerValue=-th  UpperValue=th  SaturateOnIntegerOverflow=on
  Gain : Gain  Gain=1/(1-th)
  y : Outport
  wires:
  u/1 -> Dead Zone/1
  Dead Zone/1 -> Gain/1
  Gain/1 -> y/1

== system FMS/FMS Commander/Commander/Arm/MC_Mode/Assist/Altitude/Attitude Command/Phi_CMD_TD ==
  v : Inport
  Integrator : DiscreteIntegrator  SampleTime=-1  ICPrevOutput=DiscIntNeverNeededParam  ICPrevScaledInput=DiscIntNeverNeededParam
  Integrator1 : DiscreteIntegrator  SampleTime=-1  ICPrevOutput=DiscIntNeverNeededParam  ICPrevScaledInput=DiscIntNeverNeededParam
  Subtract : Sum  Inputs=+-
  "fhan " : Subsystem  mask{r0=4*pi, h0=0.04}
      mask DialogControl ParameterGroupVar Prompt: fhan(v1,v2,r0,h0)
  v1 : Outport
  wires:
  "fhan "/1(fhan) -> Integrator/1
  Subtract/1 -> "fhan "/1(v1)
  Integrator/1 -> Integrator1/1, "fhan "/2(v2)  "v2"
  v/1 -> Subtract/2
  Integrator1/1 -> Subtract/1, v1/1

== system FMS/FMS Commander/Commander/Arm/MC_Mode/Assist/Altitude/Attitude Command/Theta_CMD_TD ==
  v : Inport
  Integrator : DiscreteIntegrator  SampleTime=-1  ICPrevOutput=DiscIntNeverNeededParam  ICPrevScaledInput=DiscIntNeverNeededParam
  Integrator1 : DiscreteIntegrator  SampleTime=-1  ICPrevOutput=DiscIntNeverNeededParam  ICPrevScaledInput=DiscIntNeverNeededParam
  Subtract : Sum  Inputs=+-
  "fhan " : Subsystem  mask{r0=4*pi, h0=0.04}
      mask DialogControl ParameterGroupVar Prompt: fhan(v1,v2,r0,h0)
  v1 : Outport
  wires:
  Integrator1/1 -> v1/1, Subtract/1
  v/1 -> Subtract/2
  Integrator/1 -> Integrator1/1, "fhan "/2(v2)  "v2"
  Subtract/1 -> "fhan "/1(v1)
  "fhan "/1(fhan) -> Integrator/1

== system FMS/FMS Commander/Commander/Arm/MC_Mode/Assist/Altitude/Heading Command/Controller ==
  motion_state : Inport
  In Bus Element : Inport  Port=2  PortName=FMS_In
  In Bus Element1 : Inport  Port=2  PortName=FMS_In
  Brake Control : Subsystem  TreatAsAtomicUnit=on
  Hold Control : Subsystem  TreatAsAtomicUnit=on
  Merge : Merge  Inputs=3
  Move Control : Subsystem  TreatAsAtomicUnit=on
  Saturation : Saturate  UpperLimit=FMS_PARAM.YAW_RATE_LIM  LowerLimit=-FMS_PARAM.YAW_RATE_LIM
  Switch Case : SwitchCase  CaseConditions={MotionState.Hold, MotionState.Brake, MotionState.Move}  ShowDefaultCase=off
  psi_rate_cmd_radPs : Outport
  wires:
  Move Control/1(psi_rate_cmd_radPs) -> Merge/3
  Brake Control/1(psi_rate_cmd_radPs) -> Merge/2
  Hold Control/1(psi_rate_cmd_radPs) -> Merge/1
  In Bus Element/1 -> Hold Control/1(FMS_In)
  Switch Case/3 -> Move Control/Action
  Switch Case/2 -> Brake Control/Action
  Switch Case/1 -> Hold Control/Action
  motion_state/1 -> Switch Case/1
  Saturation/1 -> psi_rate_cmd_radPs/1
  Merge/1 -> Saturation/1
  In Bus Element1/1 -> Move Control/1(FMS_In)

== system FMS/FMS Commander/Commander/Arm/MC_Mode/Assist/Altitude/Heading Command/Detect Movement ==
  FMS_In : Inport
  Abs : Abs
  Abs1 : Abs
  Bus Selector : BusSelector  OutputSignals=Pilot_Cmd.stick_yaw,INS_Out.r
  Compare To Constant : simulink/Logic and Bit Operations/Compare To Constant  relop=>  const=FMS_PARAM.YAW_DZ  OutDataTypeStr=boolean
  Motion State : Stateflow chart  TreatAsAtomicUnit=on
  motion_state : Outport
  wires:
  FMS_In/1 -> Bus Selector/1
  Abs1/1 -> Compare To Constant/1
  Motion State/1(state) -> motion_state/1
  Compare To Constant/1 -> Motion State/1(motion_req)
  Abs/1 -> Motion State/2(speed)
  Bus Selector/1 -> Abs1/1  "<stick_yaw>"
  Bus Selector/2 -> Abs/1  "<r>"

== system FMS/FMS Commander/Commander/Arm/MC_Mode/Assist/Position/Altitude Command/Controller ==
  motion_state : Inport
  In Bus Element : Inport  Port=2  PortName=FMS_In
  In Bus Element1 : Inport  Port=2  PortName=FMS_In
  Brake Control : Subsystem  TreatAsAtomicUnit=on
  Hold Control : Subsystem  TreatAsAtomicUnit=on
  Merge : Merge  Inputs=3
  Move Control : Subsystem  TreatAsAtomicUnit=on
  Saturation1 : Saturate  UpperLimit=FMS_PARAM.VEL_Z_LIM  LowerLimit=-FMS_PARAM.VEL_Z_LIM
  Switch Case : SwitchCase  CaseConditions={MotionState.Hold, MotionState.Brake, MotionState.Move}  ShowDefaultCase=off
  w_cmd_mPs : Outport
  wires:
  Move Control/1(w_cmd_mPs) -> Merge/3
  Brake Control/1(psi_rate_cmd_radPs) -> Merge/2
  Hold Control/1(w_cmd_mPs) -> Merge/1
  In Bus Element/1 -> Hold Control/1(FMS_In)
  Switch Case/3 -> Move Control/Action
  Switch Case/2 -> Brake Control/Action
  Switch Case/1 -> Hold Control/Action
  motion_state/1 -> Switch Case/1
  Saturation1/1 -> w_cmd_mPs/1
  Merge/1 -> Saturation1/1
  In Bus Element1/1 -> Move Control/1(FMS_In)

== system FMS/FMS Commander/Commander/Arm/MC_Mode/Assist/Position/Altitude Command/Detect Movement ==
  FMS_In : Inport
  Abs : Abs
  Abs1 : Abs
  Bus Selector : BusSelector  OutputSignals=Pilot_Cmd.stick_throttle,INS_Out.vd
  Compare To Constant : simulink/Logic and Bit Operations/Compare To Constant  relop=>  const=FMS_PARAM.THROTTLE_DZ  OutDataTypeStr=boolean
  Motion Status : Stateflow chart  TreatAsAtomicUnit=on
  motion_state : Outport
  wires:
  FMS_In/1 -> Bus Selector/1
  Abs1/1 -> Compare To Constant/1
  Motion Status/1(state) -> motion_state/1
  Compare To Constant/1 -> Motion Status/1(motion_req)
  Abs/1 -> Motion Status/2(speed)
  Bus Selector/1 -> Abs1/1  "<stick_throttle>"
  Bus Selector/2 -> Abs/1  "<vd>"

== system FMS/FMS Commander/Commander/Arm/MC_Mode/Assist/Position/Heading Command/Controller ==
  motion_state : Inport
  In Bus Element : Inport  Port=2  PortName=FMS_In
  In Bus Element1 : Inport  Port=2  PortName=FMS_In
  Brake Control : Subsystem  TreatAsAtomicUnit=on
  Hold Control : Subsystem  TreatAsAtomicUnit=on
  Merge : Merge  Inputs=3
  Move Control : Subsystem  TreatAsAtomicUnit=on
  Saturation : Saturate  UpperLimit=FMS_PARAM.YAW_RATE_LIM  LowerLimit=-FMS_PARAM.YAW_RATE_LIM
  Switch Case : SwitchCase  CaseConditions={MotionState.Hold, MotionState.Brake, MotionState.Move}  ShowDefaultCase=off
  psi_rate_cmd_radPs : Outport
  wires:
  Move Control/1(psi_rate_cmd_radPs) -> Merge/3
  Brake Control/1(psi_rate_cmd_radPs) -> Merge/2
  Hold Control/1(psi_rate_cmd_radPs) -> Merge/1
  In Bus Element/1 -> Hold Control/1(FMS_In)
  Switch Case/3 -> Move Control/Action
  Switch Case/2 -> Brake Control/Action
  Switch Case/1 -> Hold Control/Action
  motion_state/1 -> Switch Case/1
  Saturation/1 -> psi_rate_cmd_radPs/1
  Merge/1 -> Saturation/1
  In Bus Element1/1 -> Move Control/1(FMS_In)

== system FMS/FMS Commander/Commander/Arm/MC_Mode/Assist/Position/Heading Command/Detect Movement ==
  FMS_In : Inport
  Abs : Abs
  Abs1 : Abs
  Bus Selector : BusSelector  OutputSignals=Pilot_Cmd.stick_yaw,INS_Out.r
  Compare To Constant : simulink/Logic and Bit Operations/Compare To Constant  relop=>  const=FMS_PARAM.YAW_DZ  OutDataTypeStr=boolean
  Motion State : Stateflow chart  TreatAsAtomicUnit=on
  motion_state : Outport
  wires:
  FMS_In/1 -> Bus Selector/1
  Abs1/1 -> Compare To Constant/1
  Motion State/1(state) -> motion_state/1
  Compare To Constant/1 -> Motion State/1(motion_req)
  Abs/1 -> Motion State/2(speed)
  Bus Selector/1 -> Abs1/1  "<stick_yaw>"
  Bus Selector/2 -> Abs/1  "<r>"

== system FMS/FMS Commander/Commander/Arm/MC_Mode/Assist/Position/Position Command/Controller ==
  motion_state : Inport
  In Bus Element : Inport  Port=2  PortName=FMS_In
  In Bus Element1 : Inport  Port=2  PortName=FMS_In
  Hold Control : Subsystem  TreatAsAtomicUnit=on
  Merge : Merge
  Move Control : Subsystem  TreatAsAtomicUnit=on
  Saturation1 : Saturate  UpperLimit=FMS_PARAM.VEL_XY_LIM  LowerLimit=-FMS_PARAM.VEL_XY_LIM
  Switch Case : SwitchCase  CaseConditions={MotionState.Hold, [MotionState.Brake, MotionState.Move]}  ShowDefaultCase=off
  uv_cmd_mPs : Outport
  wires:
  Move Control/1(uv_cmd_mPs) -> Merge/2
  Hold Control/1(uv_cmd_mPs) -> Merge/1
  In Bus Element/1 -> Hold Control/1(FMS_In)
  Switch Case/2 -> Move Control/Action
  Switch Case/1 -> Hold Control/Action
  motion_state/1 -> Switch Case/1
  Saturation1/1 -> uv_cmd_mPs/1
  Merge/1 -> Saturation1/1
  In Bus Element1/1 -> Move Control/1(FMS_In)

== system FMS/FMS Commander/Commander/Arm/MC_Mode/Assist/Position/Position Command/Detect Movement ==
  FMS_In : Inport
  Abs1 : Abs
  Abs2 : Abs
  Add : Sum
  Bus Selector1 : BusSelector  OutputSignals=Pilot_Cmd.stick_pitch,Pilot_Cmd.stick_roll,INS_Out.vn,INS_Out.ve
  Compare To Constant : simulink/Logic and Bit Operations/Compare To Constant  relop=>  const=FMS_PARAM.ROLL_DZ  OutDataTypeStr=boolean
  Compare To Constant1 : simulink/Logic and Bit Operations/Compare To Constant  relop=>  const=FMS_PARAM.PITCH_DZ  OutDataTypeStr=boolean
  Logical Operator : Logic  Operator=OR  AllPortsSameDT=off  OutDataTypeStr=boolean
  Motion State : Stateflow chart  TreatAsAtomicUnit=on
  Sqrt : Sqrt  SaturateOnIntegerOverflow=on
  Square : Math  Operator=square  SaturateOnIntegerOverflow=on
  Square1 : Math  Operator=square  SaturateOnIntegerOverflow=on
  motion_state : Outport
  wires:
  FMS_In/1 -> Bus Selector1/1
  Add/1 -> Sqrt/1
  Square1/1 -> Add/2
  Square/1 -> Add/1
  Logical Operator/1 -> Motion State/1(motion_req)
  Compare To Constant/1 -> Logical Operator/2
  Compare To Constant1/1 -> Logical Operator/1
  Abs2/1 -> Compare To Constant1/1
  Abs1/1 -> Compare To Constant/1
  Motion State/1(state) -> motion_state/1  "pos_ms"
  Sqrt/1 -> Motion State/2(speed)  "spd"
  Bus Selector1/1 -> Abs2/1  "<stick_pitch>"
  Bus Selector1/2 -> Abs1/1  "<stick_roll>"
  Bus Selector1/3 -> Square/1  "<vn>"
  Bus Selector1/4 -> Square1/1  "<ve>"

== system FMS/FMS Commander/Commander/Arm/MC_Mode/Assist/Stabilize/Attitude Command/DeadZone ==
  u : Inport
  Dead Zone : DeadZone  LowerValue=-th  UpperValue=th  SaturateOnIntegerOverflow=on
  Gain : Gain  Gain=1/(1-th)
  y : Outport
  wires:
  Gain/1 -> y/1
  Dead Zone/1 -> Gain/1
  u/1 -> Dead Zone/1
